simulink model "Driver"  (R2026b)
settings: Solver=VariableStepAuto
undefined symbols (not defined in the file): Driver, Maneuver, Scene, Vehicle, Visual, X, xy_data_car_side, Y, Z
libraries: sm_lib x18, simulink x13, nesl_utility x5, drivingvehiclecontroller x1, autolibshared x1, $bdroot x1
(part 1 of 2)
settings Model: Creator=andrei  LastModifiedBy=andrei

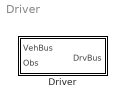
== system Driver ==
  Driver : Subsystem  Variant=on  VariantControlMode=label  VariantControl=Variant1  LabelModeActiveChoice=Closed_Loop  mask(Driver){popup_driver_type=Closed Loop}
      mask prompts: popup_driver_type "Driver"
      mask help: Models driver behavior. Open loop driver specifies positions of accelerator, brake pedal, and steering wheel. Closed loop driver compares current vehicle pose (x, y, theta) and current vehicle speed with target position and speed.
      mask init:
      | set_param(gcb,'LabelModeActiveChoice',strrep(get_param(gcb,'popup_driver_type'),' ','_'));
      settings: AttributesFormatString=%<popup_driver_type>
      mask TypeOptions popup_driver_type: Closed Loop | Closed Loop1 | Open Loop
      mask Display: disp(' ')

== system Driver/Driver ==
  "VehBus " : Inport
  Obs : Inport  Port=2
  Closed Loop : Subsystem  VariantControl=Closed_Loop
  Closed Loop1 : $bdroot/Driver/Closed Loop  SystemSampleTime=-1  VariantControl=Closed_Loop1  VariantActivationTime=update diagram  EmptyChoice=off  PassThrough=off  PassThroughVariantControl=(default)  EmptyChoiceVariantControl=(default)  AllowFlexibleInterface=on  Latency=0  AutoFrameSizeCalculation=off
  Open Loop : Subsystem  VariantControl=Open_Loop
  " DrvBus" : Outport  VectorParamsAs1DForOutWhenUnconnected=off

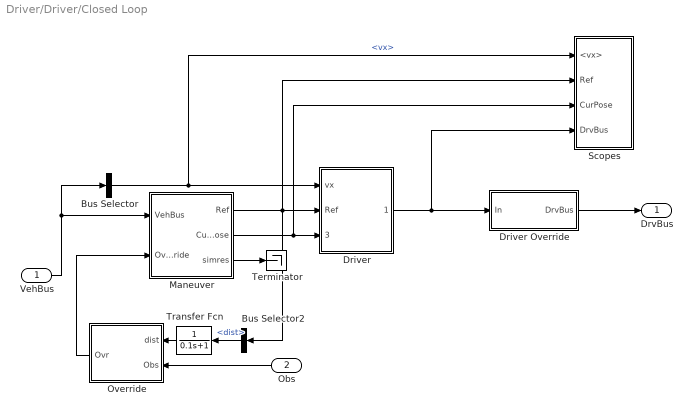
== system Driver/Driver/Closed Loop ==
  VehBus : Inport
  Obs : Inport  Port=2
  Bus Selector : BusSelector  OutputSignals=Chassis.Body.CG.vx
  Bus Selector2 : BusSelector  OutputSignals=dist
  Driver : Subsystem  mask(Driver Behavior){Driver=Driver}
      mask help: Models driver behavior to follow prescribed vehicle trajectory, including path and speed.
  Driver Override : Subsystem  Variant=on  VariantControlMode=label  VariantControl=Choice  LabelModeActiveChoice=None  mask(Override Driver Commands){popup_driver_override=None}
      mask prompts: popup_driver_override "Driver Override"
      mask help: Override closed-loop driver commands with open-loop inputs. Can be applied to steering wheel, accelerator pedal. or brake pedal.
      mask init:
      | curblk = gcb;
      | 
      | set_param(curblk,'LabelModeActiveChoice',get_param(curblk,'popup_driver_override'));
      mask TypeOptions popup_driver_override: None | Override
  Maneuver : Subsystem  mask(Maneuver Follow Trajectory){Maneuver=Maneuver, Value=Maneuver.vGain.Value, popup_window=No}
      mask prompts: Value "vGain"; popup_window "Check only window of trajectory"
      mask help: Determines target pose to follow prescribed trajectory. Prescribed trajectory is vehicle pose (x, y, theta) and speed along the path to be followed. Optional visual of target pose is also provided.
      mask init:
      | if(strcmpi(get_param(gcb,'popup_window'),'yes'))
      |     set_param([gcb '/window only'],'Value','1');
      | else
      |     set_param([gcb '/window only'],'Value','0');
      | end
      mask TypeOptions Value: Target Speed Gain/Value
      mask TypeOptions popup_window: No | Yes
  Override : Subsystem  Variant=on  VariantControlMode=label  VariantControl=Variant1  LabelModeActiveChoice=None  mask(Driver Override){popup_override_type=None}
      mask prompts: popup_override_type "Override Type"
      mask help: Optionally override driver commands based on objects in scene. For example, the state of a traffic light can override driver commands to follow a prescribed speed trajectory.
      mask init:
      | set_param(gcb,'LabelModeActiveChoice',strrep(get_param(gcb,'popup_override_type'),' ','_'));
      settings: AttributesFormatString=%<LabelModeActiveChoice>
      mask TypeOptions popup_override_type: None | Track Mallory Park Obstacle
      mask Display: disp(' ');
  Scopes : Subsystem
  Terminator : Terminator
  Transfer Fcn : TransferFcn  Denominator=[0.1 1]
  DrvBus : Outport  VectorParamsAs1DForOutWhenUnconnected=off
  wires:
  Override/1(" Ovr") -> Maneuver/2(Override)
  Bus Selector/1 -> Driver/1(vx), Scopes/1(<vx>)  "<vx>"
  VehBus/1 -> Maneuver/1(VehBus), Bus Selector/1
  Maneuver/2(CurPose) -> Driver/3(CurPose), Scopes/3(CurPose)
  Maneuver/1(Ref) -> Driver/2(Ref), Scopes/2(Ref), Bus Selector2/1
  Maneuver/3(simres) -> Terminator/1
  Driver Override/1(DrvBus) -> DrvBus/1
  Driver/1(DrvBus) -> Scopes/4(DrvBus), Driver Override/1(In)
  Transfer Fcn/1 -> Override/1("dist ")
  Bus Selector2/1 -> Transfer Fcn/1  "<dist>"
  Obs/1 -> Override/2("Obs ")

== system Driver/Driver/Open Loop ==
  VehBus : Inport
  Obs : Inport  Port=2
  Open Loop : Subsystem  mask{Maneuver=Maneuver}
      mask init:
      | X = [0 0];
      | Y = [0 0];
  Terminator : Terminator
  Terminator1 : Terminator
  DrvBus : Outport  VectorParamsAs1DForOutWhenUnconnected=off
  wires:
  Open Loop/1(DrvBus) -> DrvBus/1
  VehBus/1 -> Terminator/1
  Obs/1 -> Terminator1/1

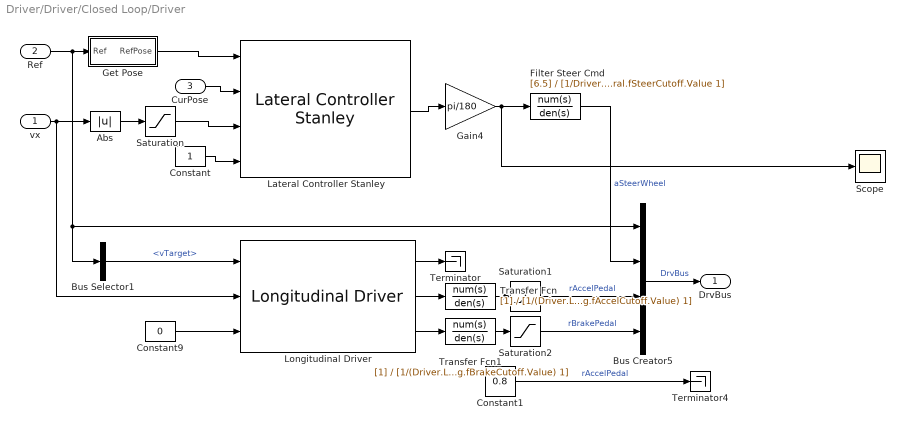
== system Driver/Driver/Closed Loop/Driver ==
  vx : Inport
  Ref : Inport  Port=2
  CurPose : Inport  Port=3
  Abs : Abs  SaturateOnIntegerOverflow=off
  Bus Creator5 : BusCreator  Inputs=4
  Bus Selector1 : BusSelector  OutputSignals=vTarget
  Constant : Constant
  Constant1 : Constant  Value=0.8
  Constant9 : Constant  Value=0
  Filter Steer Cmd : TransferFcn  Numerator=[6.5]  Denominator=[1/Driver.Lateral.fSteerCutoff.Value 1]
  Gain4 : Gain  Gain=pi/180
  Get Pose : Subsystem
  Lateral Controller Stanley : drivingvehiclecontroller/Lateral Controller Stanley  ModelType=Kinematic bicycle model  PositionGainF=0.7  PositionGainR=Driver.Lateral.Stanley.NForward.Value  YawRateGain=0.2  DelayGain=0.2  VehicleMass=1575  Lf=1.2  Lr=1.6  TireStiffness=19000  Wheelbase=1.578  MaxSteeringAngle=27
  Longitudinal Driver : autolibshared/Longitudinal Driver  extAccelOvr=off  extDecelOvr=off  extAccelHld=off  extDecelHld=off  extAccelZero=off  extDecelZero=off  cntrlType=Predictive  shftType=None  velUnits=m/s  gearOut=off  Kp=15  Ki=1  Kff=.05  Kg=.01  VehVelVec=[0 100]  KffVec=[.1 .1]  KpVec=[10 10]  KiVec=[5 5]  KgVec=[0 0]  m=320  Kpt=Driver.Long.FTractive.Value  tau=Driver.Long.tDriver.Value  L=3  aR=Driver.Long.NDragRoll.Value  bR=Driver.Long.NDragAero.Value  cR=Driver.Long.NDragAero.Value  g=Driver.Long.gGravity.Value  vnom=100  Kaw=.1  tauerr=.03  tauPt=2  GearInit=0  tShift=.1  pdlVec=[0.1 0.4 0.5 0.9]  upShftTbl=[-1 12.9375 26.4375 39.9375 51.18749999999999 62.4375 72.84375 83.25;-1 16.3125 29.8125 43.3125 54.5624 65.8125 76.78125 87.75;-1 19.6875 33.1875 46.68749999999999 57.9375 69.1875 80.71875 92.25;-1 33 52.5 77.25 100.5 138.75 161.875 185]  dwnShftTbl=[1 9.5625 23.0625 36.5625 47.8125 59.0625 68.90625 78.75;1 12.9375 26.4375 39.9375 51.18749999999999 62.4375 72.84375 83.25;1 16.3125 29.8125 43.3125 54.562499 65.8125 76.78125 87.75;1 19.6875 33.1875 46.68749999999999 57.9375 69.1875 80.71875 92.25]  tClutch=.5  tRev=.5  tPark=120  aMode=1  UpGearVec="[0  1  2  3  4  5  6  7]"  DownGearVec="[1  2  3  4  5  6  7  8]"
  Saturation : Saturate  UpperLimit=inf  LowerLimit=1e-9  ZeroCross=off
  Saturation1 : Saturate  UpperLimit=1  LowerLimit=0  ZeroCross=off
  Saturation2 : Saturate  UpperLimit=1  LowerLimit=0  ZeroCross=off
  Scope : Scope
      settings: ActiveDisplayYMinimum=-1  ActiveDisplayYMaximum=1  DataLoggingVariableName=ScopeData8
  Terminator : Terminator
  Terminator4 : Terminator
  Transfer Fcn : TransferFcn  Denominator=[1/(Driver.Long.fAccelCutoff.Value) 1]
  Transfer Fcn1 : TransferFcn  Denominator=[1/(Driver.Long.fBrakeCutoff.Value) 1]
  DrvBus : Outport  VectorParamsAs1DForOutWhenUnconnected=off
  wires:
  Gain4/1 -> Filter Steer Cmd/1, Scope/1
  Constant1/1 -> Terminator4/1  "rAccelPedal"
  Saturation2/1 -> Bus Creator5/4  "rBrakePedal"
  Saturation1/1 -> Bus Creator5/3  "rAccelPedal"
  Longitudinal Driver/2 -> Transfer Fcn/1
  Constant9/1 -> Longitudinal Driver/3
  Bus Creator5/1 -> DrvBus/1  "DrvBus"
  Bus Selector1/1 -> Longitudinal Driver/1  "<vTarget>"
  Lateral Controller Stanley/1 -> Gain4/1
  Longitudinal Driver/1 -> Terminator/1
  CurPose/1 -> Lateral Controller Stanley/2
  Longitudinal Driver/3 -> Transfer Fcn1/1
  Abs/1 -> Saturation/1
  Transfer Fcn1/1 -> Saturation2/1
  Transfer Fcn/1 -> Saturation1/1
  vx/1 -> Abs/1, Longitudinal Driver/2
  Ref/1 -> Get Pose/1(Ref), Bus Creator5/1, Bus Selector1/1
  Get Pose/1(RefPose) -> Lateral Controller Stanley/1
  Filter Steer Cmd/1 -> Bus Creator5/2  "aSteerWheel"
  Saturation/1 -> Lateral Controller Stanley/3
  Constant/1 -> Lateral Controller Stanley/4

== system Driver/Driver/Closed Loop/Driver Override ==
  In : Inport
  None : Subsystem  VariantControl=None
  Override : Subsystem  VariantControl=Override
  DrvBus : Outport

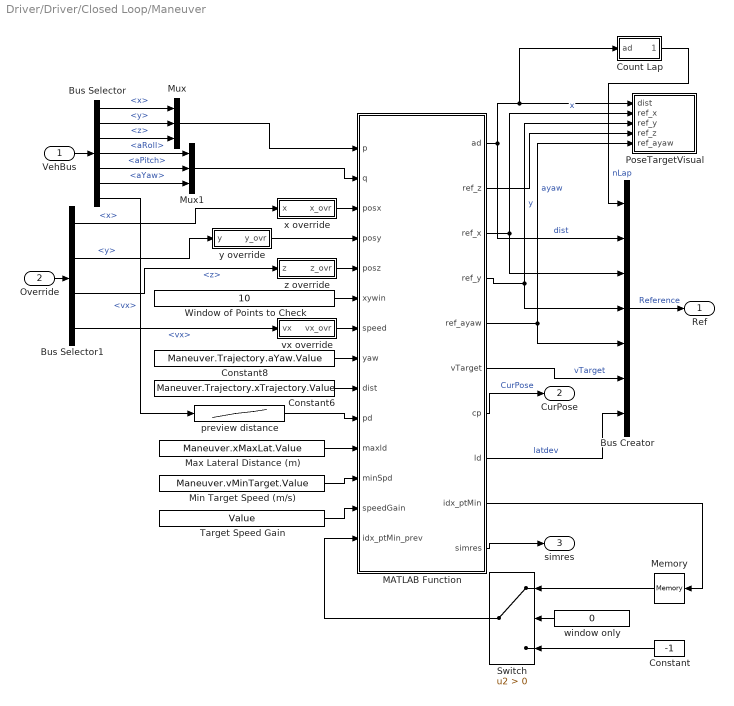
== system Driver/Driver/Closed Loop/Maneuver ==
  VehBus : Inport
  Override : Inport  Port=2
  Bus Creator : BusCreator  Inputs=7
  Bus Selector : BusSelector  OutputSignals=World.x,World.y,World.z,World.aRoll,World.aPitch,World.aYaw,Chassis.Body.CG.vx
  Bus Selector1 : BusSelector  OutputSignals=x,y,z,vx
  Constant : Constant  Value=-1
  Constant6 : Constant  Value=Maneuver.Trajectory.xTrajectory.Value
  Constant8 : Constant  Value=Maneuver.Trajectory.aYaw.Value
  Count Lap : Subsystem
  MATLAB Function : MATLAB Function  SystemSampleTime=0.1
  Max Lateral Distance (m) : Constant  Value=Maneuver.xMaxLat.Value
  Memory : Memory  InitialCondition=-1
  Min Target Speed (m/s) : Constant  Value=Maneuver.vMinTarget.Value
  Mux : Mux  Inputs=3
  Mux1 : Mux  Inputs=3
  PoseTargetVisual : Subsystem
  Switch : Switch  Criteria=u2 > Threshold  SaturateOnIntegerOverflow=off  InputSameDT=off
  Target Speed Gain : Constant  Value=Value
  Window of Points to Check : Constant  Value=10
  preview distance : Lookup_n-D  NumberOfTableDimensions=1  BreakpointsForDimension1=Maneuver.xPreview.v.Value  Table=Maneuver.xPreview.x.Value  InternalRulePriority=Speed  RndMeth=Simplest
  vx override : Subsystem
  window only : Constant  Value=0
  x override : Subsystem
  y override : Subsystem
  z override : Subsystem
  Ref : Outport  VectorParamsAs1DForOutWhenUnconnected=off
  CurPose : Outport  Port=2  VectorParamsAs1DForOutWhenUnconnected=off
  simres : Outport  Port=3  VectorParamsAs1DForOutWhenUnconnected=off
  wires:
  Count Lap/1(lapC) -> Bus Creator/1  "nLap"
  MATLAB Function/8(ld) -> Bus Creator/7  "latdev"
  Min Target Speed (m/s)/1 -> MATLAB Function/12(minSpd)
  Target Speed Gain/1 -> MATLAB Function/13(speedGain)
  Max Lateral Distance (m)/1 -> MATLAB Function/11(maxld)
  Bus Selector/1 -> Mux/1  "<x>"
  Bus Selector/6 -> Mux1/3  "<aYaw>"
  Bus Selector/4 -> Mux1/1  "<aRoll>"
  Constant8/1 -> MATLAB Function/8(yaw)
  Bus Selector/7 -> preview distance/1  "<vx>"
  Mux1/1 -> MATLAB Function/2(q)
  Bus Selector/5 -> Mux1/2  "<aPitch>"
  Constant6/1 -> MATLAB Function/9(dist)
  Mux/1 -> MATLAB Function/1(p)
  Bus Selector/3 -> Mux/3  "<z>"
  y override/1(y_ovr) -> MATLAB Function/4(posy)
  Bus Selector/2 -> Mux/2  "<y>"
  MATLAB Function/3(ref_x) -> PoseTargetVisual/2(ref_x), Bus Creator/3  "x"
  x override/1(x_ovr) -> MATLAB Function/3(posx)
  MATLAB Function/7(cp) -> CurPose/1  "CurPose"
  preview distance/1 -> MATLAB Function/10(pd)
  VehBus/1 -> Bus Selector/1
  MATLAB Function/4(ref_y) -> PoseTargetVisual/3(ref_y), Bus Creator/4  "y"
  MATLAB Function/5(ref_ayaw) -> PoseTargetVisual/5(ref_ayaw), Bus Creator/5  "ayaw"
  MATLAB Function/1(ad) -> Bus Creator/2, PoseTargetVisual/1(dist), Count Lap/1(ad)  "dist"
  Bus Creator/1 -> Ref/1  "Reference"
  MATLAB Function/6(vTarget) -> Bus Creator/6  "vTarget"
  MATLAB Function/10(simres) -> simres/1
  Window of Points to Check/1 -> MATLAB Function/6(xywin)
  MATLAB Function/9(idx_ptMin) -> Memory/1
  Switch/1 -> MATLAB Function/14(idx_ptMin_prev)
  Constant/1 -> Switch/3
  window only/1 -> Switch/2
  Memory/1 -> Switch/1
  MATLAB Function/2(ref_z) -> PoseTargetVisual/4(ref_z)
  z override/1(z_ovr) -> MATLAB Function/5(posz)
  Override/1 -> Bus Selector1/1
  Bus Selector1/4 -> vx override/1(vx)  "<vx>"
  vx override/1(vx_ovr) -> MATLAB Function/7(speed)
  Bus Selector1/3 -> z override/1(z)  "<z>"
  Bus Selector1/2 -> y override/1(y)  "<y>"
  Bus Selector1/1 -> x override/1(x)  "<x>"

== system Driver/Driver/Closed Loop/Override ==
  "dist " : Inport
  "Obs " : Inport  Port=2
  None : Subsystem  VariantControl=None  mask(No Driver Override){override=Scene.Mallory_Park_Obstacle.Override}
      mask prompts: override "Override parameters (structure)"
      mask help: Driver commands are not overridden, regardless of inputs to subsystem.
  " Ovr" : Outport  VectorParamsAs1DForOutWhenUnconnected=off

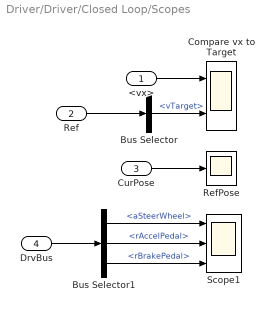
== system Driver/Driver/Closed Loop/Scopes ==
  <vx> : Inport
  Ref : Inport  Port=2
  CurPose : Inport  Port=3
  DrvBus : Inport  Port=4
  Bus Selector : BusSelector  OutputSignals=vTarget
  Bus Selector1 : BusSelector  OutputSignals=aSteerWheel,rAccelPedal,rBrakePedal
  Compare vx to Target : Scope  NumInputPorts=2
      settings: ActiveDisplayYMinimum=-4.79181  ActiveDisplayYMaximum=0.54534
  RefPose : Scope
      settings: ActiveDisplayYMinimum=-598.75829  ActiveDisplayYMaximum=469.37365
  Scope1 : Scope  NumInputPorts=3
      settings: ActiveDisplayYMinimum=-1.19495  ActiveDisplayYMaximum=0.13277  DataLoggingVariableName=ScopeData2
  wires:
  Ref/1 -> Bus Selector/1
  Bus Selector/1 -> Compare vx to Target/2  "<vTarget>"
  CurPose/1 -> RefPose/1
  Bus Selector1/3 -> Scope1/3  "<rBrakePedal>"
  <vx>/1 -> Compare vx to Target/1
  Bus Selector1/2 -> Scope1/2  "<rAccelPedal>"
  Bus Selector1/1 -> Scope1/1  "<aSteerWheel>"
  DrvBus/1 -> Bus Selector1/1

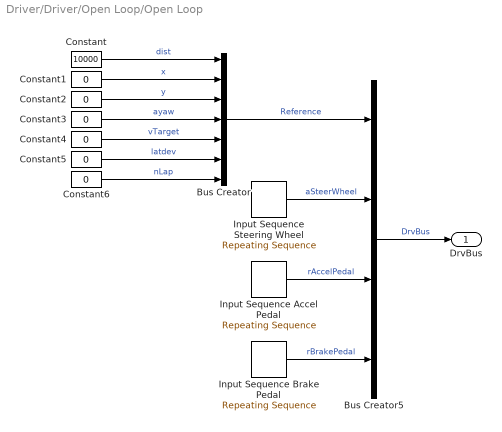
== system Driver/Driver/Open Loop/Open Loop ==
  Bus Creator : BusCreator  Inputs=7
  Bus Creator5 : BusCreator  Inputs=4
  Constant : Constant  Value=10000
  Constant{1..6} (6 alike) : Constant  Value=0
  Input Sequence Accel Pedal : simulink/Sources/Repeating Sequence  rep_seq_t=Maneuver.Accel.t.Value  rep_seq_y=Maneuver.Accel.rPedal.Value
  Input Sequence Brake Pedal : simulink/Sources/Repeating Sequence  rep_seq_t=Maneuver.Brake.t.Value  rep_seq_y=Maneuver.Brake.rPedal.Value
  "Input Sequence Steering Wheel " : simulink/Sources/Repeating Sequence  rep_seq_t=Maneuver.Steer.t.Value  rep_seq_y=Maneuver.Steer.aWheel.Value
  DrvBus : Outport  VectorParamsAs1DForOutWhenUnconnected=off
  wires:
  Bus Creator5/1 -> DrvBus/1  "DrvBus"
  Input Sequence Brake Pedal/1 -> Bus Creator5/4  "rBrakePedal"
  "Input Sequence Steering Wheel "/1 -> Bus Creator5/2  "aSteerWheel"
  Input Sequence Accel Pedal/1 -> Bus Creator5/3  "rAccelPedal"
  Constant1/1 -> Bus Creator/2  "x"
  Constant5/1 -> Bus Creator/6  "latdev"
  Constant2/1 -> Bus Creator/3  "y"
  Constant3/1 -> Bus Creator/4  "ayaw"
  Constant4/1 -> Bus Creator/5  "vTarget"
  Bus Creator/1 -> Bus Creator5/1  "Reference"
  Constant/1 -> Bus Creator/1  "dist"
  Constant6/1 -> Bus Creator/7  "nLap"

== system Driver/Driver/Closed Loop/Driver/Get Pose ==
  Ref : Inport
  Bus Selector : BusSelector  OutputSignals=x,y,ayaw
  Gain : Gain  Gain=180/pi
  Mux : Mux  Inputs=3
  RefPose : Outport  VectorParamsAs1DForOutWhenUnconnected=off
  wires:
  Bus Selector/1 -> Mux/1  "<x>"
  Ref/1 -> Bus Selector/1
  Mux/1 -> RefPose/1
  Bus Selector/2 -> Mux/2  "<y>"
  Bus Selector/3 -> Gain/1  "<ayaw>"
  Gain/1 -> Mux/3

== system Driver/Driver/Closed Loop/Driver Override/None ==
  In : Inport
  DrvBus : Outport
  wires:
  In/1 -> DrvBus/1

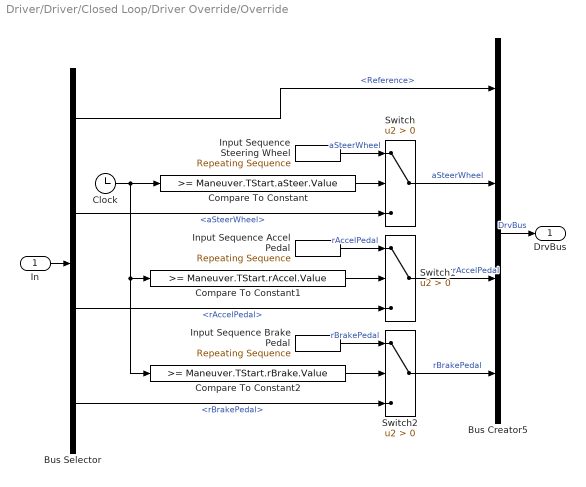
== system Driver/Driver/Closed Loop/Driver Override/Override ==
  In : Inport
  Bus Creator5 : BusCreator  Inputs=4
  Bus Selector : BusSelector  OutputSignals=Reference,aSteerWheel,rAccelPedal,rBrakePedal
  Clock : Clock
  Compare To Constant : simulink/Logic and Bit Operations/Compare To Constant  relop=>=  const=Maneuver.TStart.aSteer.Value  OutDataTypeStr=boolean
  Compare To Constant1 : simulink/Logic and Bit Operations/Compare To Constant  relop=>=  const=Maneuver.TStart.rAccel.Value  OutDataTypeStr=boolean
  Compare To Constant2 : simulink/Logic and Bit Operations/Compare To Constant  relop=>=  const=Maneuver.TStart.rBrake.Value  OutDataTypeStr=boolean
  Input Sequence Accel Pedal : simulink/Sources/Repeating Sequence  rep_seq_t=Maneuver.Accel.t.Value  rep_seq_y=Maneuver.Accel.rPedal.Value
  Input Sequence Brake Pedal : simulink/Sources/Repeating Sequence  rep_seq_t=Maneuver.Brake.t.Value  rep_seq_y=Maneuver.Brake.rPedal.Value
  Input Sequence Steering Wheel : simulink/Sources/Repeating Sequence  rep_seq_t=Maneuver.Steer.t.Value  rep_seq_y=Maneuver.Steer.aWheel.Value
  Switch : Switch  Criteria=u2 > Threshold  SaturateOnIntegerOverflow=off  InputSameDT=off
  Switch1 : Switch  Criteria=u2 > Threshold  SaturateOnIntegerOverflow=off  InputSameDT=off
  Switch2 : Switch  Criteria=u2 > Threshold  SaturateOnIntegerOverflow=off  InputSameDT=off
  DrvBus : Outport
  wires:
  Compare To Constant2/1 -> Switch2/2
  Compare To Constant1/1 -> Switch1/2
  In/1 -> Bus Selector/1
  Bus Creator5/1 -> DrvBus/1  "DrvBus"
  Bus Selector/2 -> Switch/3  "<aSteerWheel>"
  Switch/1 -> Bus Creator5/2  "aSteerWheel"
  Bus Selector/1 -> Bus Creator5/1  "<Reference>"
  Bus Selector/3 -> Switch1/3  "<rAccelPedal>"
  Switch1/1 -> Bus Creator5/3  "rAccelPedal"
  Bus Selector/4 -> Switch2/3  "<rBrakePedal>"
  Clock/1 -> Compare To Constant2/1, Compare To Constant1/1, Compare To Constant/1
  Compare To Constant/1 -> Switch/2
  Switch2/1 -> Bus Creator5/4  "rBrakePedal"
  Input Sequence Steering Wheel/1 -> Switch/1  "aSteerWheel"
  Input Sequence Accel Pedal/1 -> Switch1/1  "rAccelPedal"
  Input Sequence Brake Pedal/1 -> Switch2/1  "rBrakePedal"

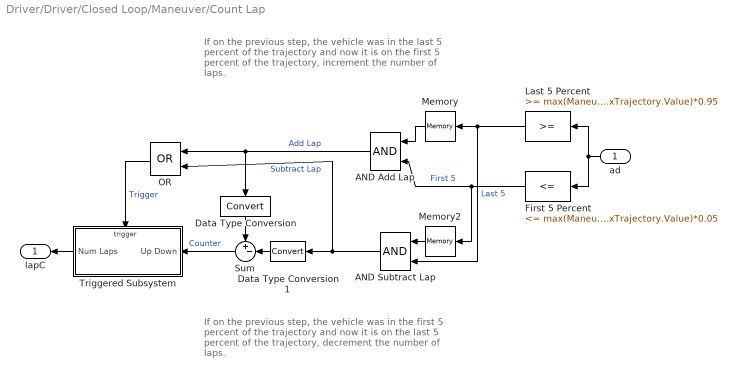
== system Driver/Driver/Closed Loop/Maneuver/Count Lap ==
  note: If on the previous step, the vehicle was in the last 5 percent of the trajectory and now it is on the first 5 percent of the trajectory, increment the number of laps.
  note: If on the previous step, the vehicle was in the first 5 percent of the trajectory and now it is on the last 5 percent of the trajectory, decrement the number of laps.
  ad : Inport
  AND Add Lap : Logic  IconShape=distinctive  AllPortsSameDT=off  OutDataTypeStr=boolean
  AND Subtract Lap : Logic  IconShape=distinctive  AllPortsSameDT=off  OutDataTypeStr=boolean
  Data Type Conversion : DataTypeConversion  SaturateOnIntegerOverflow=off  RndMeth=Floor
  Data Type Conversion1 : DataTypeConversion  SaturateOnIntegerOverflow=off  RndMeth=Floor
  First 5 Percent : simulink/Logic and Bit Operations/Compare To Constant  relop=<=  const=max(Maneuver.Trajectory.xTrajectory.Value)*0.05  OutDataTypeStr=boolean  ZeroCross=off
  Last 5 Percent : simulink/Logic and Bit Operations/Compare To Constant  relop=>=  const=max(Maneuver.Trajectory.xTrajectory.Value)*0.95  OutDataTypeStr=boolean  ZeroCross=off
  Memory : Memory  InitialCondition=false
  Memory2 : Memory  InitialCondition=false
  OR : Logic  Operator=OR  IconShape=distinctive  AllPortsSameDT=off  OutDataTypeStr=boolean
  Sum : Sum  Inputs=+-|
  Triggered Subsystem : Subsystem  TreatAsAtomicUnit=on
  lapC : Outport  VectorParamsAs1DForOutWhenUnconnected=off
  wires:
  Data Type Conversion1/1 -> Sum/2
  Data Type Conversion/1 -> Sum/1
  ad/1 -> First 5 Percent/1, Last 5 Percent/1
  Last 5 Percent/1 -> AND Subtract Lap/2, Memory/1  "Last 5"
  Triggered Subsystem/1(Num Laps) -> lapC/1
  First 5 Percent/1 -> Memory2/1, AND Add Lap/2  "First 5"
  Memory/1 -> AND Add Lap/1
  OR/1 -> Triggered Subsystem/Trigger  "Trigger"
  Memory2/1 -> AND Subtract Lap/1
  AND Add Lap/1 -> Data Type Conversion/1, OR/1  "Add Lap"
  AND Subtract Lap/1 -> OR/2, Data Type Conversion1/1  "Subtract Lap"
  Sum/1 -> Triggered Subsystem/1(Up Down)  "Counter"

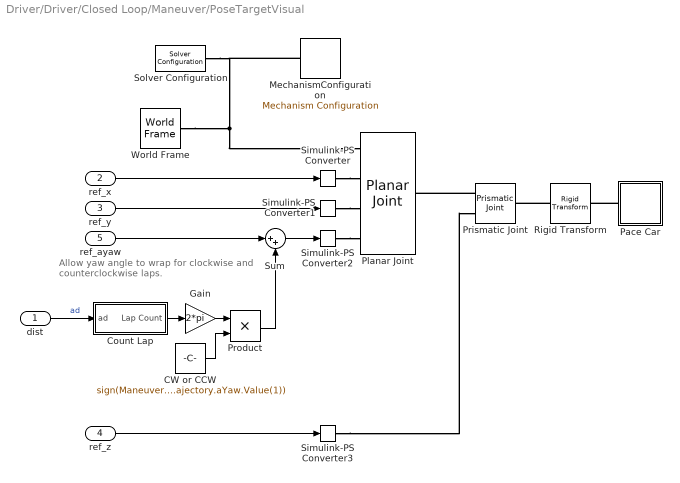
== system Driver/Driver/Closed Loop/Maneuver/PoseTargetVisual ==
  note: Allow yaw angle to wrap for
      | clockwise and counterclockwise laps.
  dist : Inport
  ref_x : Inport  Port=2
  ref_y : Inport  Port=3
  ref_z : Inport  Port=4
  ref_ayaw : Inport  Port=5
  CW or CCW : Constant  Value=sign(Maneuver.Trajectory.aYaw.Value(end)-Maneuver.Trajectory.aYaw.Value(1))
  Count Lap : Subsystem
  Gain : Gain  Gain=2*pi
  MechanismConfiguration : sm_lib/Utilities/Mechanism Configuration  UniformGravity=None  GravityVector=[0 0 -9.80665]  GravityVectorUnits=m/s^2  LinearizationDelta=0.001  JointModeTransitionNonlinearIterations=2
  Pace Car : Subsystem  mask(Car Body Geometry){whl_cutout_rad=0.5, whl_base=abs(Vehicle.Chassis.Body.sAxle1.Value(1)-Vehicle.Chassis.Body.sAxle2.Value(1)), thk_top=0.05, thk_side=0.05, car_track=Vehicle.Chassis.Body.Width.Value, offset_ref=[0 0 0.3225], extr_data_emblem_f=Visual.PaceCar.emblem.data*0.2, extr_data_emblem_r=Visual.PaceCar.emblem.data*0.2, clr_body_geo_top=Visual.PaceCar.body.clr, opc_body_geo_top=Visual.PaceCar.body.opc, clr_body_geo_left=Visual.PaceCar.body.clr, opc_body_geo_left=Visual.PaceCar.body.opc, clr_body_geo_right=Visual.PaceCar.body.clr, opc_body_geo_right=Visual.PaceCar.body.opc, clr_emblem_f=Visual.PaceCar.body.clr, opc_emblem_f=Visual.PaceCar.emblem.opc, clr_emblem_r=Visual.PaceCar.body.clr, opc_emblem_r=Visual.PaceCar.emblem.opc}
      mask prompts: whl_cutout_rad "Wheel Cutout Radius (m)"; whl_base "Wheelbase (m)"; thk_top "Top Thickness (m)"; thk_side "Side Thickness (m)"; car_track "Width (m)"; offset_ref "Offset to reference frame [xyz] (m)"; extr_data_emblem_f "Emblem Data Front [xy] (m)"; extr_data_emblem_r "Emblem Data Rear [xy] (m)"
      mask help: Creates simple car geometry. Adjusting the wheel cutout radius and wheelbase causes the profile to be adjusted. Press the Plot Profile button to see how the parameters affect the profile.
      mask init:
      | [xy_data_car_top xy_data_car_side] = Extr_Data_Car_Profile(whl_cutout_rad, whl_base,thk_top);
      mask TypeOptions extr_data_emblem_f:
      | Ornament
      | Front/ExtrusionCrossSection
      mask TypeOptions extr_data_emblem_r:
      | Ornament
      | Rear/ExtrusionCrossSection
      mask TypeOptions clr_body_geo_top: Top Surface/GraphicDiffuseColor
      mask TypeOptions opc_body_geo_top: Top Surface/GraphicOpacity
      mask TypeOptions clr_body_geo_left: Left Face/GraphicDiffuseColor
      mask TypeOptions opc_body_geo_left: Left Face/GraphicOpacity
      mask TypeOptions clr_body_geo_right: Right Face/GraphicDiffuseColor
      mask TypeOptions opc_body_geo_right: Right Face/GraphicOpacity
      mask TypeOptions clr_emblem_f:
      | Ornament
      | Front/GraphicDiffuseColor
      mask TypeOptions opc_emblem_f:
      | Ornament
      | Front/GraphicOpacity
      mask TypeOptions clr_emblem_r:
      | Ornament
      | Rear/GraphicDiffuseColor
      mask TypeOptions opc_emblem_r:
      | Ornament
      | Rear/GraphicOpacity
      mask DialogControl cont_geometry Prompt: Body Geometry
      mask DialogControl push_plot_profile Prompt: Plot Profile
      mask DialogControl push_plot_profile Callback:
      | v = get_param(gcb,'MaskWSVariables');
      | getMaskValue = containers.Map({v.Name}',{v.Value}');
      | evalin('base',...
      |     sprintf('Extr_Data_Car_Profile(%s,%s,%s,''%s'');',...
      |     num2str(getMaskValue('whl_cutout_rad')),...
      |     num2str(getMaskValue('whl_base')),...
      |     num2str(getMaskValue('thk_top')),'plot'));
      mask DialogControl cont_emblem Prompt: Emblem
      mask DialogControl cont_vis Prompt: Visualization
      mask DialogControl text_vis_clr Prompt: Color [RGB]
      mask DialogControl text_vis_opc Prompt: Opac. (0-1)
      mask DialogControl text_vis_top Prompt: Top
      mask DialogControl text_vis_left Prompt: Left Side
      mask DialogControl text_vis_right Prompt: Right Side
      mask DialogControl text_vis_emblem_f Prompt: Emblem Front
      mask DialogControl text_vis_emblem_r Prompt: Emblem Rear
      mask Display: image('sm_car_bodygeometry_sedan.png');
  Planar Joint : sm_lib/Joints/Planar Joint  JointMode=Normal  CompositeWrenchDir=FollowerOnBase  CompositeWrenchFrame=BaseFrame  SenseConstraintForce=off  SenseConstraintTorque=off  SenseTotalForce=off  SenseTotalTorque=off  PxPositionTargetSpecify=off  PxPositionTargetPriority=High  PxPositionTargetValue=0  PxPositionTargetValueUnits=m  PxVelocityTargetSpecify=off  PxVelocityTargetPriority=High  PxVelocityTargetValue=0  PxVelocityTargetValueUnits=m/s  PxEquilibriumPosition=0  PxEquilibriumPositionUnits=m  PxSpringStiffness=1  PxSpringStiffnessUnits=N/m  PxDampingCoefficient=1  PxDampingCoefficientUnits=N/(m/s)  PxLowerLimitSpecify=off  PxLowerLimitBound=-1  PxLowerLimitBoundUnits=m  PxLowerLimitStiffness=1e6  PxLowerLimitStiffnessUnits=N/m  PxLowerLimitDamping=1e3  PxLowerLimitDampingUnits=N/(m/s)  PxLowerLimitTransitionRegionWidth=1e-4  PxLowerLimitTransitionRegionWidthUnits=m  PxUpperLimitSpecify=off  PxUpperLimitBound=1  PxUpperLimitBoundUnits=m  PxUpperLimitStiffness=1e6  PxUpperLimitStiffnessUnits=N/m  PxUpperLimitDamping=1e3  PxUpperLimitDampingUnits=N/(m/s)  PxUpperLimitTransitionRegionWidth=1e-4  PxUpperLimitTransitionRegionWidthUnits=m  PxTorqueActuationMode=ComputedTorque  PxMotionActuationMode=InputMotion  PxSensePosition=off  PxSenseVelocity=off  PxSenseAcceleration=off  PxSenseTorqueForce=off  PxSenseLowerLimitTorqueForce=off  PxSenseUpperLimitTorqueForce=off  PyPositionTargetSpecify=off  PyPositionTargetPriority=High  PyPositionTargetValue=0  PyPositionTargetValueUnits=m  PyVelocityTargetSpecify=off  PyVelocityTargetPriority=High  PyVelocityTargetValue=0  PyVelocityTargetValueUnits=m/s  PyEquilibriumPosition=0  PyEquilibriumPositionUnits=m  PySpringStiffness=1  PySpringStiffnessUnits=N/m  PyDampingCoefficient=1  PyDampingCoefficientUnits=N/(m/s)  PyLowerLimitSpecify=off  PyLowerLimitBound=-1  PyLowerLimitBoundUnits=m  PyLowerLimitStiffness=1e6  PyLowerLimitStiffnessUnits=N/m  PyLowerLimitDamping=1e3  PyLowerLimitDampingUnits=N/(m/s)  PyLowerLimitTransitionRegionWidth=1e-4  PyLowerLimitTransitionRegionWidthUnits=m  PyUpperLimitSpecify=off  PyUpperLimitBound=1  PyUpperLimitBoundUnits=m  PyUpperLimitStiffness=1e6  PyUpperLimitStiffnessUnits=N/m  PyUpperLimitDamping=1e3  PyUpperLimitDampingUnits=N/(m/s)  PyUpperLimitTransitionRegionWidth=1e-4  PyUpperLimitTransitionRegionWidthUnits=m  PyTorqueActuationMode=ComputedTorque  PyMotionActuationMode=InputMotion  PySensePosition=off  PySenseVelocity=off  PySenseAcceleration=off  PySenseTorqueForce=off  PySenseLowerLimitTorqueForce=off  PySenseUpperLimitTorqueForce=off  RzPositionTargetSpecify=off  RzPositionTargetPriority=High  RzPositionTargetValue=0  RzPositionTargetValueUnits=deg  RzVelocityTargetSpecify=off  RzVelocityTargetPriority=High  RzVelocityTargetValue=0  RzVelocityTargetValueUnits=deg/s  RzEquilibriumPosition=0  RzEquilibriumPositionUnits=deg  RzSpringStiffness=1  RzSpringStiffnessUnits=N*m/deg  RzDampingCoefficient=1  RzDampingCoefficientUnits=N*m/(deg/s)  RzLowerLimitSpecify=off  RzLowerLimitBound=-90  RzLowerLimitBoundUnits=deg  RzLowerLimitStiffness=1e4  RzLowerLimitStiffnessUnits=N*m/deg  RzLowerLimitDamping=10  RzLowerLimitDampingUnits=N*m/(deg/s)  RzLowerLimitTransitionRegionWidth=0.1  RzLowerLimitTransitionRegionWidthUnits=deg  RzUpperLimitSpecify=off  RzUpperLimitBound=90  RzUpperLimitBoundUnits=deg  RzUpperLimitStiffness=1e4  RzUpperLimitStiffnessUnits=N*m/deg  RzUpperLimitDamping=10  RzUpperLimitDampingUnits=N*m/(deg/s)  RzUpperLimitTransitionRegionWidth=0.1  RzUpperLimitTransitionRegionWidthUnits=deg  RzTorqueActuationMode=ComputedTorque  RzMotionActuationMode=InputMotion  RzSensePosition=off  RzSenseVelocity=off  RzSenseAcceleration=off  RzSenseTorqueForce=off  RzSenseLowerLimitTorqueForce=off  RzSenseUpperLimitTorqueForce=off
  Prismatic Joint : sm_lib/Joints/Prismatic Joint  JointMode=Normal  CompositeWrenchDir=FollowerOnBase  CompositeWrenchFrame=BaseFrame  SenseConstraintForce=off  SenseConstraintTorque=off  SenseTotalForce=off  SenseTotalTorque=off  PositionTargetSpecify=off  PositionTargetPriority=High  PositionTargetValue=0  PositionTargetValueUnits=m  VelocityTargetSpecify=off  VelocityTargetPriority=High  VelocityTargetValue=0  VelocityTargetValueUnits=m/s  EquilibriumPosition=0  EquilibriumPositionUnits=m  SpringStiffness=0  SpringStiffnessUnits=N/m  DampingCoefficient=0  DampingCoefficientUnits=N/(m/s)  LowerLimitSpecify=off  LowerLimitBound=-1  LowerLimitBoundUnits=m  LowerLimitStiffness=1e6  LowerLimitStiffnessUnits=N/m  LowerLimitDamping=1e3  LowerLimitDampingUnits=N/(m/s)  LowerLimitTransitionRegionWidth=1e-4  LowerLimitTransitionRegionWidthUnits=m  UpperLimitSpecify=off  UpperLimitBound=1  UpperLimitBoundUnits=m  UpperLimitStiffness=1e6  UpperLimitStiffnessUnits=N/m  UpperLimitDamping=1e3  UpperLimitDampingUnits=N/(m/s)  UpperLimitTransitionRegionWidth=1e-4  UpperLimitTransitionRegionWidthUnits=m  TorqueActuationMode=ComputedTorque  MotionActuationMode=InputMotion  SensePosition=off  SenseVelocity=off  SenseAcceleration=off  SenseTorqueForce=off  SenseLowerLimitTorqueForce=off  SenseUpperLimitTorqueForce=off
  Product : Product
  Rigid Transform : sm_lib/Frames and Transforms/Rigid Transform  RotationMethod=None  FollAlignAxisA=+X  BaseAlignAxisA=+Y  FollAlignAxisB=+Y  BaseAlignAxisB=+Z  RotationStandardAxis=+Z  RotationAngle=0.0  RotationAngleUnits=deg  RotationArbitraryAxis=[0 0 1]  RotationSequenceAxes=FollowerAxes  RotationSequence=XYX  RotationSequenceAngles=[0 0 0]  RotationSequenceAnglesUnits=deg  RotationMatrix=[1 0 0; 0 1 0; 0 0 1]  Quaternion=[1 0 0 0]  TranslationMethod=Cartesian  TranslationCartesianOffset=[0 0 0.1]  TranslationCartesianOffsetUnits=m  TranslationStandardAxis=+Z  TranslationStandardOffset=0  TranslationStandardOffsetUnits=m  TranslationROffset=0  TranslationROffsetUnits=m  TranslationThetaOffset=0  TranslationThetaOffsetUnits=deg  TranslationZOffset=0  TranslationZOffsetUnits=m
  Simulink-PS Converter : nesl_utility/Simulink-PS Converter  PhysicalDomain=network_engine_domain  SubClassName=ps_input  LeftPortType=input  RightPortType=output  PseudoPeriodic=off  Frequencies=[]  NoiseDistribution=none  NoiseParameters=[]  Unit=1  AffineConversion=off  FilteringAndDerivatives=filter  SimscapeFilterOrder=2  InputFilterTimeConstant=0.1  UdotUserProvided=0
  Simulink-PS Converter1 : nesl_utility/Simulink-PS Converter  PhysicalDomain=network_engine_domain  SubClassName=ps_input  LeftPortType=input  RightPortType=output  PseudoPeriodic=off  Frequencies=[]  NoiseDistribution=none  NoiseParameters=[]  Unit=1  AffineConversion=off  FilteringAndDerivatives=filter  SimscapeFilterOrder=2  InputFilterTimeConstant=0.1  UdotUserProvided=0
  Simulink-PS Converter2 : nesl_utility/Simulink-PS Converter  PhysicalDomain=network_engine_domain  SubClassName=ps_input  LeftPortType=input  RightPortType=output  PseudoPeriodic=off  Frequencies=[]  NoiseDistribution=none  NoiseParameters=[]  Unit=rad  AffineConversion=off  FilteringAndDerivatives=filter  SimscapeFilterOrder=2  InputFilterTimeConstant=0.1  UdotUserProvided=0
  Simulink-PS Converter3 : nesl_utility/Simulink-PS Converter  PhysicalDomain=network_engine_domain  SubClassName=ps_input  LeftPortType=input  RightPortType=output  PseudoPeriodic=off  Frequencies=[]  NoiseDistribution=none  NoiseParameters=[]  Unit=1  AffineConversion=off  FilteringAndDerivatives=filter  SimscapeFilterOrder=2  InputFilterTimeConstant=0.1  UdotUserProvided=0
  Solver Configuration : nesl_utility/Solver Configuration  PhysicalDomain=network_engine_domain  SubClassName=solver  LeftPortType=input  RightPortType=generic  Tones=[]  Harmonics=[]  SimulateNoise=off  Profile=off  UseLocalSampling=off  EnableSwitchedLinearOptims=on  FrequencyDomain=off  UseCCode=off  RelTol=0.001  AbsTol=1e-06  MinStep=1e-09  ToWorkspace=off  RevertToSquareIcSolve=off  NumHomotopyIterations=100  PhasorMode=off  PhasorModeNumHarmonics=1  ConsistencySolver=NEWTON_XTOL_AFTER_FTOL  CanonicalOrdering=UNORDERED  OptimizeIntermediates=UNOPTIMIZED  MulticoreSolverChoice=BACKWARD_EULER  IndexReductionMethod=DerivativeReplacement  DoDC=off  ResidualTolerance=1e-9  ConsistencyTolSource=GLOBAL  ConsistencyAbsTol=0.001  ConsistencyRelTol=0.001  ConsistencyTolFactor=0.001  UseLocalSolver=off  LocalSolverChoice=NE_BACKWARD_EULER_ADVANCER  ResolveIndetEquations=on  FunctionEvalNumThread=1  LocalSolverSampleTime=0.001  DoFixedCost=off  MaxNonlinIter=5  MaxModeIter=2  ComputeImpulses=off  ImpulseIterations=2  LinearAlgebra=Sparse  LinearAlgebraNumThread=0  EquationFormulation=NE_TIME_EF  DelaysMemoryBudget=1024  AutomaticFiltering=on  FilteringTimeConstant=0.001  PartitionStorageMethod=AS_NEEDED  PartitionMemoryBudget=1024  PartitionMethod=FAST  MultibodyUseLocalSolver=off  MultibodyLocalSolverChoice=ODE1  MultibodyLocalSolverSampleTime=0.001
  Sum : Sum  Inputs=|++
  World Frame : sm_lib/Frames and Transforms/World Frame
  wires:
  CW or CCW/1 -> Product/2
  Gain/1 -> Product/1
  Sum/1 -> Simulink-PS Converter2/1
  Product/1 -> Sum/2
  Count Lap/1(Lap Count) -> Gain/1
  dist/1 -> Count Lap/1(ad)  "ad"
  ref_ayaw/1 -> Sum/1
  ref_y/1 -> Simulink-PS Converter1/1
  ref_x/1 -> Simulink-PS Converter/1
  ref_z/1 -> Simulink-PS Converter3/1
  connections:
  Pace Car/LConn1 -- Rigid Transform/RConn1
  Simulink-PS Converter/RConn1 -- Planar Joint/LConn2
  Simulink-PS Converter2/RConn1 -- Planar Joint/LConn4
  Rigid Transform/LConn1 -- Prismatic Joint/RConn1
  Simulink-PS Converter1/RConn1 -- Planar Joint/LConn3
  World Frame/RConn1 -- Planar Joint/LConn1 -- MechanismConfiguration/RConn1 -- Solver Configuration/RConn1
  Prismatic Joint/LConn1 -- Planar Joint/RConn1
  Simulink-PS Converter3/RConn1 -- Prismatic Joint/LConn2

== system Driver/Driver/Closed Loop/Maneuver/vx override ==
  note: Override speed signal using
      | gain (to set to zero) and/or with an
      | offset (for passing maneuver).
  vx : Inport
  Bus Selector2 : BusSelector  OutputSignals=offset,gain
  Constant5 : Constant  Value=Maneuver.Trajectory.vx.Value
  Product : Product
  Sum : Sum  Inputs=++|
  vx_ovr : Outport  VectorParamsAs1DForOutWhenUnconnected=off
  wires:
  Bus Selector2/1 -> Sum/1  "<offset>"
  Product/1 -> Sum/2
  Constant5/1 -> Product/2
  Sum/1 -> vx_ovr/1
  Bus Selector2/2 -> Product/1  "<gain>"
  vx/1 -> Bus Selector2/1

== system Driver/Driver/Closed Loop/Maneuver/x override ==
  note: Override speed signal using
      | gain (to set to zero) and/or with an
      | offset (for passing maneuver).
  x : Inport
  Bus Selector2 : BusSelector  OutputSignals=offset,gain
  Constant3 : Constant  Value=Maneuver.Trajectory.x.Value
  Product : Product
  Sum : Sum  Inputs=++|
  x_ovr : Outport  VectorParamsAs1DForOutWhenUnconnected=off
  wires:
  x/1 -> Bus Selector2/1
  Bus Selector2/2 -> Product/1  "<gain>"
  Sum/1 -> x_ovr/1
  Constant3/1 -> Product/2
  Product/1 -> Sum/2
  Bus Selector2/1 -> Sum/1  "<offset>"

== system Driver/Driver/Closed Loop/Maneuver/y override ==
  note: Override speed signal using
      | gain (to set to zero) and/or with an
      | offset (for passing maneuver).
  y : Inport
  Bus Selector2 : BusSelector  OutputSignals=offset,gain
  Constant4 : Constant  Value=Maneuver.Trajectory.y.Value
  Product : Product
  Sum : Sum  Inputs=++|
  y_ovr : Outport  VectorParamsAs1DForOutWhenUnconnected=off
  wires:
  Bus Selector2/1 -> Sum/1  "<offset>"
  Product/1 -> Sum/2
  Constant4/1 -> Product/2
  Sum/1 -> y_ovr/1
  Bus Selector2/2 -> Product/1  "<gain>"
  y/1 -> Bus Selector2/1

== system Driver/Driver/Closed Loop/Maneuver/z override ==
  note: Override speed signal using
      | gain (to set to zero) and/or with an
      | offset (for passing maneuver).
  z : Inport
  Bus Selector2 : BusSelector  OutputSignals=offset,gain
  Constant1 : Constant  Value=Maneuver.Trajectory.z.Value
  Product : Product
  Sum : Sum  Inputs=++|
  z_ovr : Outport  VectorParamsAs1DForOutWhenUnconnected=off
  wires:
  z/1 -> Bus Selector2/1
  Bus Selector2/2 -> Product/1  "<gain>"
  Sum/1 -> z_ovr/1
  Constant1/1 -> Product/2
  Product/1 -> Sum/2
  Bus Selector2/1 -> Sum/1  "<offset>"

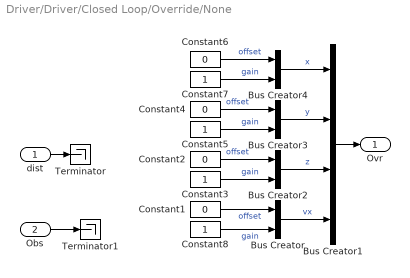
== system Driver/Driver/Closed Loop/Override/None ==
  dist : Inport
  Obs : Inport  Port=2
  Bus Creator{,2..4} (4 alike) : BusCreator  Inputs=2
  Bus Creator1 : BusCreator  Inputs=4
  Constant{1..2,4,6} (4 alike) : Constant  Value=0
  Constant{3,5,7..8} (4 alike) : Constant
  Terminator : Terminator
  Terminator1 : Terminator
  Ovr : Outport  VectorParamsAs1DForOutWhenUnconnected=off
  wires:
  dist/1 -> Terminator/1
  Obs/1 -> Terminator1/1
  Bus Creator1/1 -> Ovr/1
  Constant1/1 -> Bus Creator/1  "offset"
  Constant8/1 -> Bus Creator/2  "gain"
  Constant6/1 -> Bus Creator4/1  "offset"
  Constant7/1 -> Bus Creator4/2  "gain"
  Constant5/1 -> Bus Creator3/2  "gain"
  Constant4/1 -> Bus Creator3/1  "offset"
  Constant3/1 -> Bus Creator2/2  "gain"
  Bus Creator2/1 -> Bus Creator1/3  "z"
  Constant2/1 -> Bus Creator2/1  "offset"
  Bus Creator3/1 -> Bus Creator1/2  "y"
  Bus Creator/1 -> Bus Creator1/4  "vx"
  Bus Creator4/1 -> Bus Creator1/1  "x"

== system Driver/Driver/Closed Loop/Maneuver/Count Lap/Triggered Subsystem ==
  Up Down : Inport
  Trigger : TriggerPort  VariantControl=Variant  ZeroCross=off
  Memory : Memory  InheritSampleTime=on
  Sum : Sum  Inputs=|++
  Num Laps : Outport  VectorParamsAs1DForOutWhenUnconnected=off
  wires:
  Up Down/1 -> Sum/2
  Sum/1 -> Num Laps/1, Memory/1
  Memory/1 -> Sum/1

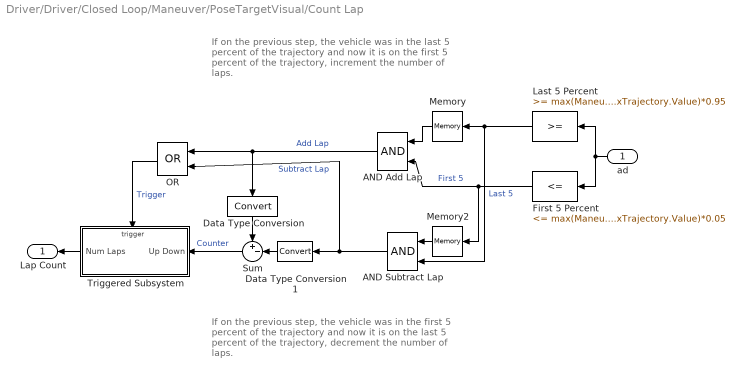
== system Driver/Driver/Closed Loop/Maneuver/PoseTargetVisual/Count Lap ==
  note: If on the previous step, the vehicle was in the first 5 percent of the trajectory and now it is on the last 5 percent of the trajectory, decrement the number of laps.
  note: If on the previous step, the vehicle was in the last 5 percent of the trajectory and now it is on the first 5 percent of the trajectory, increment the number of laps.
  ad : Inport
  AND Add Lap : Logic  IconShape=distinctive  AllPortsSameDT=off  OutDataTypeStr=boolean
  AND Subtract Lap : Logic  IconShape=distinctive  AllPortsSameDT=off  OutDataTypeStr=boolean
  Data Type Conversion : DataTypeConversion  SaturateOnIntegerOverflow=off  RndMeth=Floor
  Data Type Conversion1 : DataTypeConversion  SaturateOnIntegerOverflow=off  RndMeth=Floor
  First 5 Percent : simulink/Logic and Bit Operations/Compare To Constant  relop=<=  const=max(Maneuver.Trajectory.xTrajectory.Value)*0.05  OutDataTypeStr=boolean  ZeroCross=off
  Last 5 Percent : simulink/Logic and Bit Operations/Compare To Constant  relop=>=  const=max(Maneuver.Trajectory.xTrajectory.Value)*0.95  OutDataTypeStr=boolean  ZeroCross=off
  Memory : Memory  InitialCondition=false
  Memory2 : Memory  InitialCondition=false
  OR : Logic  Operator=OR  IconShape=distinctive  AllPortsSameDT=off  OutDataTypeStr=boolean
  Sum : Sum  Inputs=+-|
  Triggered Subsystem : Subsystem  TreatAsAtomicUnit=on
  Lap Count : Outport  VectorParamsAs1DForOutWhenUnconnected=off
  wires:
  Sum/1 -> Triggered Subsystem/1(Up Down)  "Counter"
  AND Subtract Lap/1 -> Data Type Conversion1/1, OR/2  "Subtract Lap"
  AND Add Lap/1 -> OR/1, Data Type Conversion/1  "Add Lap"
  Memory2/1 -> AND Subtract Lap/1
  OR/1 -> Triggered Subsystem/Trigger  "Trigger"
  Memory/1 -> AND Add Lap/1
  First 5 Percent/1 -> AND Add Lap/2, Memory2/1  "First 5"
  Triggered Subsystem/1(Num Laps) -> Lap Count/1
  Last 5 Percent/1 -> Memory/1, AND Subtract Lap/2  "Last 5"
  ad/1 -> Last 5 Percent/1, First 5 Percent/1
  Data Type Conversion/1 -> Sum/1
  Data Type Conversion1/1 -> Sum/2
